simulink model "ElectricVehicleThermalManagementWithHeatPump_2026a_version"  (R2026a)
settings: Solver=VariableStepAuto  StopTime=3600  AbsTol=1e-3
PreLoadFcn:
  | init_nmpc
InitFcn:
  | init_nmpc
model workspace: external: MATLAB File ElectricVehicleThermalManagementWithHeatPumpParameters.m (data not in the file)
values from neighbouring files (symbols this model uses):
  battery_C1_LUT = [1913.6 12447 30609 ... (first row only)    [ElectricVehicleThermalManagementWithHeatPumpParameters.m]
  battery_capacity_LUT = [280.081 276.25 276.392]    [ElectricVehicleThermalManagementWithHeatPumpParameters.m]
  battery_cell_cp = 795    [ElectricVehicleThermalManagementWithHeatPumpParameters.m]
  battery_cell_mass = 2.5    [ElectricVehicleThermalManagementWithHeatPumpParameters.m]
  battery_Em_LUT = [3.4966 3.5057 3.5148 ... (first row only)    [ElectricVehicleThermalManagementWithHeatPumpParameters.m]
  battery_N_cells = 20    [ElectricVehicleThermalManagementWithHeatPumpParameters.m]
  battery_Qe_init = 0    [ElectricVehicleThermalManagementWithHeatPumpParameters.m]
  battery_R0_LUT = [0.0117 0.0085 0.009 ... (first row only)    [ElectricVehicleThermalManagementWithHeatPumpParameters.m]
  battery_R1_LUT = [0.0109 0.0029 0.0013 ... (first row only)    [ElectricVehicleThermalManagementWithHeatPumpParameters.m]
  battery_SOC_LUT = [0; 0.1; 0.25; 0.5; 0.75; 0.9; 1]    [ElectricVehicleThermalManagementWithHeatPumpParameters.m]
  battery_T_init = -5    [ElectricVehicleThermalManagementWithHeatPumpParameters.m]
  battery_temperature_LUT = [5 20 40]    [ElectricVehicleThermalManagementWithHeatPumpParameters.m]
  cabin_duct_area = 0.04    [ElectricVehicleThermalManagementWithHeatPumpParameters.m]
  cabin_T_init = -5    [ElectricVehicleThermalManagementWithHeatPumpParameters.m]
  chiller_area_primary = 0.43982297150257105    (= 0.439822971503)    [ElectricVehicleThermalManagementWithHeatPumpParameters.m]
  chiller_N_baffles = 3    [ElectricVehicleThermalManagementWithHeatPumpParameters.m]
  chiller_N_tubes = 100    [ElectricVehicleThermalManagementWithHeatPumpParameters.m]
  chiller_tube_D = 0.0035    [ElectricVehicleThermalManagementWithHeatPumpParameters.m]
  chiller_tube_L = 0.4    [ElectricVehicleThermalManagementWithHeatPumpParameters.m]
  chiller_wall_conductivity = 240    [ElectricVehicleThermalManagementWithHeatPumpParameters.m]
  chiller_wall_thickness = 0.0001    [ElectricVehicleThermalManagementWithHeatPumpParameters.m]
  cond_evap_air_area_flow = 0.3906    [ElectricVehicleThermalManagementWithHeatPumpParameters.m]
  cond_evap_air_area_primary = 1.4834999999999998    (= 1.4835)    [ElectricVehicleThermalManagementWithHeatPumpParameters.m]
  cond_evap_W = 0.015    [ElectricVehicleThermalManagementWithHeatPumpParameters.m]
  cond_evap_wall_conductivity = 240    [ElectricVehicleThermalManagementWithHeatPumpParameters.m]
  cond_evap_wall_thickness = 0.0001    [ElectricVehicleThermalManagementWithHeatPumpParameters.m]
  coolant_channel_D = 0.0092    [ElectricVehicleThermalManagementWithHeatPumpParameters.m]
  coolant_pipe_D = 0.019    [ElectricVehicleThermalManagementWithHeatPumpParameters.m]
  coolant_T_init = -5    [ElectricVehicleThermalManagementWithHeatPumpParameters.m]
  coolant_tank_area = 0.0121    [ElectricVehicleThermalManagementWithHeatPumpParameters.m]
  coolant_tank_volume = 1.25    [ElectricVehicleThermalManagementWithHeatPumpParameters.m]
  coolant_valve_D_ratio_max = 0.95    [ElectricVehicleThermalManagementWithHeatPumpParameters.m]
  coolant_valve_D_ratio_min = 0.001    [ElectricVehicleThermalManagementWithHeatPumpParameters.m]
  coolant_valve_displacement = 0.0063    [ElectricVehicleThermalManagementWithHeatPumpParameters.m]
  coolant_valve_S_max = 0.0053    [ElectricVehicleThermalManagementWithHeatPumpParameters.m]
  evaporator_air_area_flow = 0.12    [ElectricVehicleThermalManagementWithHeatPumpParameters.m]
  evaporator_air_area_primary = 0.4323    [ElectricVehicleThermalManagementWithHeatPumpParameters.m]
  evaporator_W = 0.015    [ElectricVehicleThermalManagementWithHeatPumpParameters.m]
  evaporator_wall_conductivity = 240    [ElectricVehicleThermalManagementWithHeatPumpParameters.m]
  evaporator_wall_thickness = 0.0001    [ElectricVehicleThermalManagementWithHeatPumpParameters.m]
  expansion_valve_D_ratio_max = 0.9    [ElectricVehicleThermalManagementWithHeatPumpParameters.m]
  hex_area_primary = 0.070371675440411369    (= 0.0703716754404)    [ElectricVehicleThermalManagementWithHeatPumpParameters.m]
  hex_N_tubes = 64    [ElectricVehicleThermalManagementWithHeatPumpParameters.m]
  hex_tube_D = 0.0035    [ElectricVehicleThermalManagementWithHeatPumpParameters.m]
  hex_wall_conductivity = 240    [ElectricVehicleThermalManagementWithHeatPumpParameters.m]
  hex_wall_thickness = 0.0001    [ElectricVehicleThermalManagementWithHeatPumpParameters.m]
  inner_cond_air_area_flow = 0.1953    [ElectricVehicleThermalManagementWithHeatPumpParameters.m]
  inner_cond_air_area_primary = 0.99520000000000008    (= 0.9952)    [ElectricVehicleThermalManagementWithHeatPumpParameters.m]
  inner_cond_W = 0.02    [ElectricVehicleThermalManagementWithHeatPumpParameters.m]
  inner_cond_wall_conductivity = 240    [ElectricVehicleThermalManagementWithHeatPumpParameters.m]
  inner_cond_wall_thickness = 0.0001    [ElectricVehicleThermalManagementWithHeatPumpParameters.m]
  pump_speed_max = 1000    [ElectricVehicleThermalManagementWithHeatPumpParameters.m]
  radiator_air_area_flow = 0.097499999999999989    (= 0.0975)    [ElectricVehicleThermalManagementWithHeatPumpParameters.m]
  radiator_air_area_primary = 0.43687499999999996    (= 0.436875)    [ElectricVehicleThermalManagementWithHeatPumpParameters.m]
  radiator_W = 0.015    [ElectricVehicleThermalManagementWithHeatPumpParameters.m]
  radiator_wall_conductivity = 240    [ElectricVehicleThermalManagementWithHeatPumpParameters.m]
  radiator_wall_thickness = 0.0001    [ElectricVehicleThermalManagementWithHeatPumpParameters.m]
  refrigerant_p_init = 0.25    [ElectricVehicleThermalManagementWithHeatPumpParameters.m]
  refrigerant_pipe_D = 0.01    [ElectricVehicleThermalManagementWithHeatPumpParameters.m]
  refrigerant_valve_D_ratio_max = 0.95    [ElectricVehicleThermalManagementWithHeatPumpParameters.m]
  refrigerant_valve_displacement = 0.005    [ElectricVehicleThermalManagementWithHeatPumpParameters.m]
libraries: fl_lib x227, nesl_utility x162, SimscapeFluids_lib x30, LiBatteryElements_lib x16, slpidlib x3, SignalEditorBlockLib x1
(part 13 of 13)

== matlab function ElectricVehicleThermalManagementWithHeatPump_2026a_version/Controls/MPCControllerBlock/MPCController ==
  data: u_cmd output; x_meas input; Tamb_C input; Tref_K input; clntInvTout_K_meas input; clntBatTin_K_meas input; dcdcQ input; motQ input; invQ input; condEvapAirMf input; batImeas input; info output
function [u_cmd, info] = MPCController_step( ...
    x_meas, ...                         % [nx x 1] measured/estimated states (physical units)
    Tamb_C, ...                         % [1 x 1] ambient in degC
    Tref_K, ...                         % [1 x 1] cabin air reference in K
    clntInvTout_K_meas, ...             % [1 x 1] from plant (K)
    clntBatTin_K_meas, ...              % [1 x 1] from plant (K)
    dcdcQ, motQ, invQ, ...              % [1 x 1] loads (W)
    condEvapAirMf, ...                  % [1 x 1] kg/s
    batImeas)                           % [1 x 1] A
% MPCController_step
% ---------------------------------------------------------
% Simulink usage (continuous plant + discrete MPC):
% - Put MATLAB Function block calling this function in a subsystem with Ts=1
% - ZOH(Ts=1) on u_cmd into continuous plant
% - Rate Transition (to Ts=1) for feedback signals into this block
% - Add Unit Delay(Ts=1) on x_meas path if you get algebraic loop warnings
%
% IMPORTANT:
% This is a "one-step NMPC solve" function. It builds the solver once (persistent),
% then solves once per call and returns the first control move.
%
% NOTE:
% This code keeps your NMPC formulation structure, but to make it deployable in
% a MATLAB Function block, it removes:
% - clc/clear/close
% - any for-loops over ksim (closed-loop simulation loop)
% - any plant rollout inside controller (plant is Simulink)
% ---------------------------------------------------------

%#ok<*NASGU>
%#ok<*AGROW>

% import casadi.*

%% ===================== Persistent objects ============================
persistent built ...
    solver F Uord packParams idx_cmdPS ...
    dt M h N nx nu np ...
    umin umax xmin xmax ...
    Sx SxInv Su SuInv ...
    w_cost w_all p_all g lbg ubg lbw ubw ...
    n_w nX nU nSd idxSdyn idxSy idxSx_lo idxSx_hi ...
    Xsym Usym Sdynsym Sysym Sx_losym Sx_hisym ...
    prev_w_opt prev_lam_x prev_lam_g prev_Pk ...
    inputInit ...
    Stuned resampled ...
    ns_ic idx_ic_slack ...
    USE_FIXED_U USE_SCALING ...
    Tref_default ...
    Gfun

if isempty(built)
    %% =============================== Setup ===============================
    % addpath('C:\Prashant\Prashant\Phd\casadi-3.7.1-windows64-matlab2018b');

    % load('tuning_data_10.mat', 'resampled');
    % tunedVarsFile = 'tunedVariables_minus5_minus10_New.mat';
    % Stuned = load(tunedVarsFile);
    resampled = evalin('base','resampled');
    Stuned    = evalin('base','Stuned');

    [F, Uord, ~, packParams] = create_dynamics_nmpc();
    idx_cmdPS = get_idx_cmdPS(Uord);

    %% ====================== Problem sizes & settings =====================
    dt    = 1.0;     % controller sample time [s]
    M     = 1;       % RK4 sub-steps per sample
    h     = dt/M;
    N     = 30;      % prediction horizon [steps]

    USE_FIXED_U = false;
    USE_SCALING = true;

    %% ============================= Dimensions ============================
    nx = 9;
    nu = numel(Uord.inputSignal);

    %% ====================== Control input bounds =========================
    umin = [    0;   0;    100;   100;   0];
    umax = [ 6000; 0.15; 1000; 1000; 4000];

    %% ====================== State bounds (physical) ======================
    Tmin      = 10 + 273.15;   % K
    Tmax      = 75 + 273.15;   % K
    Pmin      = 0.1e5;         % Pa
    Pmax      = 6e6;           % Pa
    Tmax_cab  = 40 + 273.15;   % K
    Tmin_cab  = 15 + 273.15;  % K
    Tbmin     = 10 + 273.15;   % K
    Tbmax     = 50 + 273.15;   % K

    % [motT; invT; dcdcT; SOC; batT; p_in; p_out; cabIntT; cabAirT]
    xmin = [Tmin; Tmin; Tmin; 0.01; Tbmin; Pmin; Pmin; Tmin_cab; Tmin_cab];
    xmax = [Tmax; Tmax; Tmax; 1.0;  Tbmax; Pmax; Pmax; Tmax_cab; Tmax_cab];

    %% ============================= Scaling ===============================
    sx_data = [max(xmin(1),xmax(1));
               max(xmin(2),xmax(2));
               max(xmin(3),xmax(3));
               max(xmin(4),xmax(4));
               max(xmin(5),xmax(5));
               max(xmin(6),xmax(6));
               max(xmin(7),xmax(7));
               max(xmin(8),xmax(8));
               max(xmin(9),xmax(9))];

    su_data = [ ...
      max(umax(1), max(resampled.compNrpm));
      max(umax(2), max(resampled.cabAirMfIn));
      max(umax(3), max(resampled.motPumpNrpm));
      max(umax(4), max(resampled.motPumpNrpm));
      umax(5)];

    if USE_SCALING
        sx = sx_data(:);
        su = su_data(:);
    else
        sx = ones(nx,1);
        su = ones(nu,1);
    end

    Sx    = diag(sx);
    SxInv = diag(1./sx);
    Su    = diag(su);
    SuInv = diag(1./su);

    physX = @(Xs) Sx*Xs; %#ok<NASGU>

    %% ========================== Weights ==================================
    w = struct();
    w.cab        = 1e1;
    w.cabInt     = 1;
    w.energy     = 1e-3;
    w.du         = 1;
    w.term       = 0.1;
    w.ySlack     = 1e3;
    w.stateSlack = 1e3;

    pwrEstMax   = 11.0e3;
    Q_phys      = zeros(nx);
    Q_phys(9,9) = w.cab;
    Q_s         = Sx.' * Q_phys * Sx;
    R_s         = diag([1e-2, 1e-2, 1e-2, 1e-2, 5e-2]);
    Rd_s        = w.du * eye(nu);

    lambda_du0 = 1;
    lambda_duN = 0.5;
    lambda_du  = linspace(lambda_du0, lambda_duN, N);

    %% ===================== NLP decision variables ========================
    Xsym    = casadi.SX.sym('X',    nx, N+1);    % scaled states
    Sdynsym = casadi.SX.sym('Sdyn', nx, N);      % dynamic slacks (scaled)
    Usym    = casadi.SX.sym('U',    nu, N);      % scaled inputs
    Sysym   = casadi.SX.sym('S_y',  3,  N);      % inequality slacks (free in your script)

    idx_ic_slack = [1; 2; 3; 5; 8; 9];
    ns_ic        = numel(idx_ic_slack);
    Sx_losym     = casadi.SX.sym('Sx_lo', ns_ic, N+1);
    Sx_hisym     = casadi.SX.sym('Sx_hi', ns_ic, N+1);

    % Parameters (physical)
    p_x0          = casadi.SX.sym('p_x0',   nx, 1);
    p_Tref        = casadi.SX.sym('p_Tref', 1,  N+1);

    % ---- pack stage params size using one sample ----
    % We will determine np after first thermalLogic call at runtime too,
    % but here we build a dummy np by doing a "local" numeric call once.
    % (We do a safe default and then overwrite np later if needed.)
    % We'll set np after creating p_sample below.

    % We'll define Pstage later after np is known.
    % For building the NLP we need np now => do a dummy call:
    Tamb0 = -10;
    x0_dummy = [ ...
        20+273.15; 20+273.15; 20+273.15; 0.8; 20+273.15; ...
        2e5; 3e6; 20+273.15; 20+273.15];
    inputInit0.envT          = Tamb0 + 273.15;
    inputInit0.clntInvTout_K = Tamb0 + 273.15;
    inputInit0.clntBatTin_K  = Tamb0 + 273.15;
    inputInit0.compN         = 0;
    inputInit0.pumpN         = 100;
    inputInit0.prevMode      = 0;
    inputInit0.heaterPwr     = 0;

    heat0.dcdcQ         = 0;
    heat0.motQ          = 0;
    heat0.invQ          = 0;
    heat0.condEvapAirMf = 0.05;
    heat0.batImeas      = 0;
    heat0.superHeat     = 2;

    tuneS0 = prepParaVec(x0_dummy, Tamb0, Stuned.tunedVariables);
    [ctrl0, est0] = thermalLogicAndEstimation(x0_dummy, inputInit0, heat0);
    p_sample      = packParams(est0, ctrl0, tuneS0);
    np            = numel(p_sample);

    Pstage        = casadi.SX.sym('Pstage', np, N);
    p_u_last_phys = casadi.SX.sym('p_u_last_phys', nu, 1);

    % Terminal terms: keep them but lightweight default P=I, xT=x0, uT=u_last
    p_xT = casadi.SX.sym('p_xT', nx, 1);
    p_uT = casadi.SX.sym('p_uT', nu, 1);
    p_P  = casadi.SX.sym('p_P',  nx*nx, 1);   % vec(P)

    p_all = vertcat(p_x0, p_Tref(:), Pstage(:), p_xT, p_uT, p_P, p_u_last_phys);

    %% ============================ Objective/Constraints ==================
    w_cost = 0;
    g      = {};
    lbg    = [];
    ubg    = [];

    % Reference in scaled space
    Xref_s      = casadi.SX.zeros(nx, N+1);
    Xref_s(9,:) = p_Tref / Sx(9,9);

    % IC equality: X(:,1) = p_x0
    r0_phys   = Sx*Xsym(:,1) - p_x0;
    r0_scaled = SxInv * r0_phys;
    for i = 1:nx
        g{end+1} = r0_scaled(i);
        lbg      = [lbg; 0];
        ubg      = [ubg; 0];
    end

    % Slack penalties
    w_cost = w_cost + w.ySlack * sum1(Sysym(:).^2);
    w_cost = w_cost + w.stateSlack * ( sum1(Sx_losym(:).^2) + sum1(Sx_hisym(:).^2) );

    % Some constants used in your constraints
    clntLow  = -51+273.15;
    clntHigh = 121+273.15;

    rho_dyn2   = 5e3;
    rho_dyn1   = 1e1;

    % Dynamics + stage cost
    for k = 1:N
        xk_phys = Sx*Xsym(:,k);
        pk      = Pstage(:,k);
        Uk_phys = Su*Usym(:,k);

        % RK4
        xtmp = xk_phys;
        for j = 1:M
            [xdot1, ~, ~] = F(xtmp,               Uk_phys, pk);
            [xdot2, ~, ~] = F(xtmp + 0.5*h*xdot1, Uk_phys, pk);
            [xdot3, ~, ~] = F(xtmp + 0.5*h*xdot2, Uk_phys, pk);
            [xdot4, ~, ~] = F(xtmp +     h*xdot3, Uk_phys, pk);
            xtmp = xtmp + h/6*(xdot1 + 2*xdot2 + 2*xdot3 + xdot4);
        end

        [~, ~, pwr] = F(xtmp, Uk_phys, pk);

        % Dynamics constraints
        rk_scaled = SxInv * (Sx*Xsym(:,k+1) - xtmp);
        g{end+1}  = rk_scaled - Sdynsym(:,k);
        lbg       = [lbg; zeros(nx,1)];
        ubg       = [ubg; zeros(nx,1)];

        % Dynamic slack penalties + power
        eps_s   = 1e-5;
        Sdyn_k  = Sdynsym(:,k);
        w_cost  = w_cost + rho_dyn2*sumsqr(Sdyn_k) + rho_dyn1*sum1(sqrt(Sdyn_k.^2 + eps_s)) + pwr./pwrEstMax;

        % State tracking
        eXk = Xsym(:,k) - Xref_s(:,k);
        w_cost = w_cost + eXk.'*Q_s*eXk;

        % Parallel/serial mode constraint: mPS*(U3-U4)=0
        mPS = Pstage(idx_cmdPS, k);
        g{end+1} = mPS * (Usym(3,k) - Usym(4,k));
        lbg      = [lbg; 0];
        ubg      = [ubg; 0];

        % Input penalties + slew penalties
        Uk_s = Usym(:,k);
        w_cost = w_cost + Uk_s.' * R_s * Uk_s;

        if k == 1
            dUk_s = Usym(:,1) - (SuInv * p_u_last_phys);
        else
            dUk_s = Usym(:,k) - Usym(:,k-1);
        end
        w_cost = w_cost + lambda_du(k) * (dUk_s.' * Rd_s * dUk_s);

        % Algebraic outputs for your constraints
        [~, yavg_k, ~] = F(xtmp, Uk_phys, pk);
        innerCondRefToutK = yavg_k(10);
        innerCondAirTinK  = yavg_k(27);
        htxClntToutK      = yavg_k(6);
        refTempCompInK    = yavg_k(14);
        invClntToutK      = yavg_k(1);
        motClntToutK      = yavg_k(2);
        dcdcClntToutK     = yavg_k(5);
        heaterClntToutK   = yavg_k(7);
        heaterClntTInK    = yavg_k(30);

        Sy1k = Sysym(1,k);
        Sy2k = Sysym(2,k);
        Sy3k = Sysym(3,k);

        % innerCondRefToutK >= innerCondAirTinK (with slack)
        g{end+1} = innerCondRefToutK - innerCondAirTinK + Sy1k;
        lbg      = [lbg; 0];
        ubg      = [ubg; inf];

        % heater deltaT constraint
        dT_heater_max = 18;
        g{end+1} = heaterClntToutK - heaterClntTInK;
        lbg      = [lbg; -inf];
        ubg      = [ubg; dT_heater_max];

        % superheat-ish constraint (your #3)
        g{end+1} = (Pstage(38,k) + 2) - refTempCompInK + Sy3k;
        lbg      = [lbg; -2];
        ubg      = [ubg; 10];

        % coolant bounds
        g{end+1} = htxClntToutK;    lbg=[lbg;clntLow];  ubg=[ubg;clntHigh];
        g{end+1} = heaterClntToutK; lbg=[lbg;clntLow];  ubg=[ubg;clntHigh];
        g{end+1} = invClntToutK;    lbg=[lbg;clntLow];  ubg=[ubg;clntHigh];
        g{end+1} = motClntToutK;    lbg=[lbg;clntLow];  ubg=[ubg;clntHigh];
        g{end+1} = dcdcClntToutK;   lbg=[lbg;clntLow];  ubg=[ubg;clntHigh];
    end

    % Soft bounds over horizon for selected states
    for k = 1:(N+1)
        xk_phys = Sx*Xsym(:,k);
        for j = 1:ns_ic
            i   = idx_ic_slack(j);
            slo = Sx_losym(j,k);
            shi = Sx_hisym(j,k);

            g{end+1} = xmin(i) - xk_phys(i) - slo;   lbg=[lbg;-inf]; ubg=[ubg;0];
            g{end+1} = xk_phys(i) - xmax(i) - shi;   lbg=[lbg;-inf]; ubg=[ubg;0];
        end
    end

    % Terminal cost: (X(N+1)-xT)'*P*(X(N+1)-xT) + small tie-to-uT
    Pmat  = reshape(p_P, nx, nx);
    eXN   = Xsym(:,N+1) - (SxInv*p_xT);
    w_cost = w_cost + eXN.'*Pmat*eXN;
    uT_s   = SuInv * p_uT;
    w_cost = w_cost + 1e-3 * (Usym(:,N) - uT_s).'*R_s*(Usym(:,N) - uT_s);

    % Pack decision variables
    w_all = [Xsym(:); Usym(:); Sdynsym(:); Sysym(:); Sx_losym(:); Sx_hisym(:)];

    % Bounds
    lbw = -inf(size(w_all));
    ubw = +inf(size(w_all));

    % Hard state box bounds (scaled) for all nodes (then relaxed on slacked indices)
    xmin_s = SxInv * xmin;
    xmax_s = SxInv * xmax;
    for k = 1:(N+1)
        i0 = (k-1)*nx;
        lbw(i0 + (1:nx)) = xmin_s;
        ubw(i0 + (1:nx)) = xmax_s;
    end

    % Relax slacked temperature states to very wide hard bounds
    Tlo_hard = (-60 + 273.15);
    Thi_hard = (140 + 273.15);
    for k = 1:(N+1)
        i0 = (k-1)*nx;
        for kk = 1:ns_ic
            ii = idx_ic_slack(kk);
            lbw(i0 + ii) = Tlo_hard / sx(ii);
            ubw(i0 + ii) = Thi_hard / sx(ii);
        end
    end

    % Input bounds (scaled)
    umin_s = SuInv * umin;
    umax_s = SuInv * umax;
    offU = numel(Xsym(:));
    for k = 1:N
        u0 = offU + (k-1)*nu;
        lbw(u0 + (1:nu)) = umin_s;
        ubw(u0 + (1:nu)) = umax_s;
    end

    % Index layout
    nX   = numel(Xsym(:));
    nU   = numel(Usym(:));
    nSd  = nx*N;
    idxSdyn  = nX + nU + (1:nSd);

    nSy   = 3*N;
    idxSy = nX + nU + nSd + (1:nSy);

    nSx      = ns_ic*(N+1);
    idxSx_lo = nX + nU + nSd + nSy + (1:nSx);
    idxSx_hi = nX + nU + nSd + nSy + nSx + (1:nSx);

    % Bounds for Sx slacks
    lbw(idxSx_lo) = 0; ubw(idxSx_lo) = inf;
    lbw(idxSx_hi) = 0; ubw(idxSx_hi) = inf;

    % Bounds for S_y (your script allows negative, but you clamp later)
    lbw(idxSy) = -1000; ubw(idxSy) = 1000;

    % Bounds for Sdyn: allow free (you were not strictly bounding in scaled case)
    lbw(idxSdyn) = -inf;
    ubw(idxSdyn) =  inf;

    % Constraint function for debug (optional)
    Gfun = casadi.Function('Gfun', {w_all, p_all}, {vertcat(g{:})});

    % NLP
    prob = struct('f', w_cost, 'x', w_all, 'g', vertcat(g{:}), 'p', p_all);

    % Solver options (your robust-ish setup)
    opts = struct;
    opts.error_on_fail      = false;
    opts.print_time         = false;
    opts.ipopt.max_iter     = 2000;
    opts.ipopt.tol          = 1e-3;
    opts.ipopt.constr_viol_tol  = 1e-5;
    opts.ipopt.dual_inf_tol     = 1e-3;
    opts.ipopt.compl_inf_tol    = 1e-3;
    opts.ipopt.hessian_approximation = 'exact';
    opts.ipopt.linear_solver     = 'mumps';
    opts.ipopt.mu_strategy       = 'adaptive';
    opts.ipopt.print_level       = 0;   % set 5 if you want logs (but Simulink will spam)
    opts.calc_lam_p              = true;

    solver = casadi.nlpsol('solver', 'ipopt', prob, opts);

    % Persistent memory init
    prev_w_opt = [];
    prev_lam_x = [];
    prev_lam_g = [];

    inputInit.envT          = (Tamb_C + 273.15);
    inputInit.clntInvTout_K = (Tamb_C + 273.15);
    inputInit.clntBatTin_K  = (Tamb_C + 273.15);
    inputInit.compN         = 0;
    inputInit.pumpN         = 100;
    inputInit.prevMode      = 0;
    inputInit.heaterPwr     = 0;

    prev_Pk = repmat(p_sample, 1, N);

    Tref_default = 294.15;

    built = true;
end

%% ===================== Per-step MPC solve ============================
% Update supervisor “memory” from plant (Option P1)
inputInit.clntInvTout_K = clntInvTout_K_meas;
inputInit.clntBatTin_K  = clntBatTin_K_meas;
inputInit.envT          = Tamb_C + 273.15;

% Build horizon measurement struct (simple: hold current across horizon)
heatMeasured_k.dcdcQ         = repmat(dcdcQ, N, 1);
heatMeasured_k.motQ          = repmat(motQ,  N, 1);
heatMeasured_k.invQ          = repmat(invQ,  N, 1);
heatMeasured_k.condEvapAirMf = repmat(max(condEvapAirMf,1e-5), N, 1);
heatMeasured_k.batImeas      = repmat(max(batImeas,1e-3), N, 1);
heatMeasured_k.superHeat     = 2;

% Tune + supervisor/estimation
tuneS = prepParaVec(x_meas, Tamb_C, Stuned.tunedVariables);
[ctrl, est] = thermalLogicAndEstimation(x_meas, inputInit, heatMeasured_k);

% Pack stage params Pk
Pk = zeros(np, N);
for i = 1:N
    est_i = est;

    % overwrite stage-varying measured quantities if fields exist
    if isfield(est_i,'condEvapAirMf'), est_i.condEvapAirMf = heatMeasured_k.condEvapAirMf(i); end
    if isfield(est_i,'batImeas'),      est_i.batImeas      = heatMeasured_k.batImeas(i);      end
    if isfield(est_i,'motQmeas'),      est_i.motQmeas      = heatMeasured_k.motQ(i);          end
    if isfield(est_i,'invQmeas'),      est_i.invQmeas      = heatMeasured_k.invQ(i);          end
    if isfield(est_i,'dcdcQmeas'),     est_i.dcdcQmeas     = heatMeasured_k.dcdcQ(i);         end
    if isfield(est_i,'superheatK'),    est_i.superheatK    = heatMeasured_k.superHeat;        end

    pk_col = packParams(est_i, ctrl, tuneS);
    if ~all(isfinite(pk_col))
        pk_col = prev_Pk(:,i);
    end
    Pk(:,i) = pk_col;
end
prev_Pk = Pk;

% Reference path
if isempty(Tref_K) || ~isfinite(Tref_K)
    Tref_K = Tref_default;
end
Tref_path = Tref_K * ones(N+1,1);

% Terminal placeholders (lightweight but keeps your p_all format consistent)
xT    = x_meas;
uT    = [inputInit.compN; 0.05; inputInit.pumpN; inputInit.pumpN; inputInit.heaterPwr];
Pterm = eye(nx);

% Previous applied u (persistent)
persistent u_last
if isempty(u_last)
    u_last = uT;
end

% pvec must match p_all = [x0; Tref; Pstage(:); xT; uT; vec(P); u_last]
pvec = [x_meas; Tref_path; Pk(:); xT; uT; Pterm(:); u_last];

% Build warm start w0
w0 = zeros(n_w,1);

% states init guess: keep constant (scaled)
Xs0 = repmat(SxInv*x_meas, 1, N+1);
w0(1:nX) = Xs0(:);

% inputs init guess: keep last u (scaled)
Us0 = repmat(SuInv*u_last, 1, N);
w0(nX + (1:nU)) = Us0(:);

% slacks init guess: zeros but make soft-bound slacks feasible
w0(idxSdyn)  = 0;
w0(idxSy)    = 0;

% compute soft slacks for current X guess
Xphys0 = Sx * reshape(w0(1:nX), nx, N+1);
Sx_lo0 = zeros(ns_ic, N+1);
Sx_hi0 = zeros(ns_ic, N+1);
for kk = 1:(N+1)
    for j = 1:ns_ic
        ii = idx_ic_slack(j);
        Sx_lo0(j,kk) = max(0, xmin(ii) - Xphys0(ii,kk));
        Sx_hi0(j,kk) = max(0, Xphys0(ii,kk) - xmax(ii));
    end
end
w0(idxSx_lo) = Sx_lo0(:);
w0(idxSx_hi) = Sx_hi0(:);

% Shift warm start from previous solve if available
if ~isempty(prev_w_opt)
    w0 = shift_warm_start_full(prev_w_opt, w0, nx, nu, N, nX, nU, idxSdyn, idxSy, idxSx_lo, idxSx_hi);
end

% Solve
args = {'x0', w0, ...
        'lbx', lbw, 'ubx', ubw, ...
        'lbg', lbg, 'ubg', ubg, ...
        'p',   pvec};

if ~isempty(prev_lam_x), args(end+1:end+2) = {'lam_x0', prev_lam_x}; end
if ~isempty(prev_lam_g), args(end+1:end+2) = {'lam_g0', prev_lam_g}; end

sol = solver(args{:});
st  = solver.stats();

w_opt = full(sol.x);

% Extract first move
U_opt_s = reshape(w_opt(nX + (1:nU)), nu, N);
u_cmd   = Su * U_opt_s(:,1);

% Update warm-start memory
prev_w_opt = w_opt;
if isfield(sol,'lam_x'), prev_lam_x = full(sol.lam_x); else, prev_lam_x = []; end
if isfield(sol,'lam_g'), prev_lam_g = full(sol.lam_g); else, prev_lam_g = []; end

% Update controller memory for next call
inputInit.compN     = u_cmd(1);
inputInit.pumpN     = u_cmd(3);
inputInit.heaterPwr = u_cmd(5);
if isfield(ctrl,'thermalMode')
    inputInit.prevMode = ctrl.thermalMode;
end
u_last = u_cmd;

% Info
info.success = logical(st.success);
if isfield(st,'iter_count'), info.iter = double(st.iter_count); else, info.iter = NaN; end
if isfield(st,'return_status'), info.status = string(st.return_status); else, info.status = ""; end
info.obj = full(sol.f);

end

%% ============================ Helpers ===============================

function w0_next = shift_warm_start_full(prev_w_opt, w0, nx, nu, N, nX, nU, idxSdyn, idxSy, idxSx_lo, idxSx_hi)
    % shift X
    Xs  = reshape(prev_w_opt(1:nX), nx, N+1);
    Xs_shift = [Xs(:,2:end), Xs(:,end)];
    w0_next = w0;
    w0_next(1:nX) = Xs_shift(:);

    % shift U
    Us = reshape(prev_w_opt(nX + (1:nU)), nu, N);
    Us_shift = [Us(:,2:end), Us(:,end)];
    w0_next(nX + (1:nU)) = Us_shift(:);

    % shift Sdyn
    Sd = reshape(prev_w_opt(idxSdyn), nx, N);
    Sd_shift = [Sd(:,2:end), Sd(:,end)];
    w0_next(idxSdyn) = Sd_shift(:);

    % keep Sy, Sx_lo, Sx_hi
    w0_next(idxSy)    = prev_w_opt(idxSy);
    w0_next(idxSx_lo) = prev_w_opt(idxSx_lo);
    w0_next(idxSx_hi) = prev_w_opt(idxSx_hi);
end

function idx = get_idx_cmdPS(Uord)
    names = [Uord.estimatedParams(:); Uord.controlOut(:); Uord.tunePara(:)];
    idx   = find(strcmp(names, 'cmdParallelSerial'), 1);
    if isempty(idx)
        error('cmdParallelSerial not found in packParams order.');
    end
end

== matlab function ElectricVehicleThermalManagementWithHeatPump_2026a_version/Scenario/Power Demand/MATLAB Function ==
  data: OCV output; negSide output; speed_kph input; acceleration_current input size=1; road_grade input; lossTq output; lossInv output; lossDCDC output; battery_current output; Total_power output; U_lo input; U_hi input; power_motor_electrical_input output; blowerVF input; motPumpPwr input; SOC input; batTemp input; prevBatTemp input
function [OCV, negSide, lossTq, lossInv, lossDCDC, battery_current, Total_power, power_motor_electrical_input] = pwrEstimation(speed_kph, acceleration_current, road_grade, U_lo, U_hi, blowerVF, motPumpPwr, SOC, batTemp, prevBatTemp)
% =========================================================================
% Electric Motor and Battery Estimation Model (Simulink MATLAB Function)
% =========================================================================
% This function estimates:
%   - Electric motor torque and speed
%   - Motor, inverter, and DC-DC converter power losses
%   - Battery power demand and current using an Equivalent Circuit Model (ECM)
%
% -------------------------------------------------------------------------
% Author        : Prashant Lokur
% Affiliation   : Chalmers University of Technology
% Contact       : lokur@chalmers.se
% Created       : 2024
%
% Copyright (c) 2024 Prashant Lokur
% All rights reserved.
%
% This code is intended for academic and research use only.
% Redistribution and use in source and binary forms, with or without
% modification, are permitted provided that the above attribution is retained.
%
% For inquiries regarding licensing for commercial or industrial applications,
% please contact the author.

% This function estimates:
%   - Electric motor torque and speed
%   - Losses in motor, inverter, and DC-DC converter
%   - Battery current using an Equivalent Circuit Model (ECM)
% 
% Inputs:
%   speed_kph         - Vehicle speed (km/h)
%   acceleration_current - Vehicle acceleration (m/s^2)
%   road_grade        - Road slope in percentage (%)
%   U_lo, U_hi        - Low and high voltages of the DCDC converter (V)
%   blowerVF          - Blower voltage fraction (0 to 1)
%   motPumpPwr        - Motor pump power consumption (W)
%   SOC               - Battery State of Charge (0 to 1)
%   batTemp           - Current battery temperature (°C)
%   prevBatTemp       - Previous battery temperature used if current is invalid
%
% Outputs:
%   OCV                      - Battery open circuit voltage (V)
%   negSide                  - Intermediate calculation: -4*P_demand*R0 (for diagnostics)
%   power_motor_mechanical_output - Power at the motor shaft (W)
%   lossTq                  - Motor loss (W)
%   lossInv                 - Inverter loss (W)
%   lossDCDC                - DC-DC converter loss (W)
%   battery_current         - Estimated battery current (A)
%   Total_power             - Total battery power demand (W)
%   power_motor_electrical_input - Motor electrical input power (W)

% =========================================================================
% SECTION 1: Data Preprocessing and Constants
% =========================================================================

% Replace invalid battery temperature with previous value
if batTemp < -50 || batTemp > 150 || isnan(batTemp)
    batTemp = prevBatTemp;
end

% Constants
g = 9.81;                 % Gravity (m/s^2)
rho_air = 1.225;          % Air density (kg/m^3)
Crr = 0.015;              % Rolling resistance coefficient
Cd = 0.3;                 % Drag coefficient
wheel_radius = 0.3;       % Wheel radius (m)
gear_ratio = 8;           % Gear ratio (motor speed / wheel speed)
gear_efficiency = 0.98;   % Gear efficiency
vehicle_mass = 1200;      % Vehicle mass (kg)
frontal_area = 2;         % Frontal area (m^2)

% Convert speed to m/s
speed_mps = speed_kph * 1000 / 3600;
theta_road = atan(road_grade / 100);

% =========================================================================
% SECTION 2: Force and Power Calculations
% =========================================================================

F_rr = Crr * vehicle_mass * g * cos(theta_road);                  % Rolling resistance
F_drag = 0.5 * rho_air * Cd * frontal_area * speed_mps^2;         % Aerodynamic drag
F_gravity = vehicle_mass * g * sin(theta_road);                   % Grade force
F_inertia = vehicle_mass * acceleration_current;                  % Inertial force
F_total = F_rr + F_drag + F_gravity + F_inertia;                  % Total traction force

power_wheel = F_total * speed_mps;                                % Power at the wheels

omega_motor_rad_s = (speed_mps / wheel_radius) * gear_ratio;      % Motor speed (rad/s)
omega_motor_rpm_out = omega_motor_rad_s * (60 / (2 * pi));        % Motor speed (RPM)

torque_wheel = F_total * wheel_radius;                            % Wheel torque
torque_motor_out = torque_wheel / (gear_ratio * gear_efficiency); % Motor torque

% =========================================================================
% SECTION 3: Motor Loss Estimation
% =========================================================================

persistent MotorLossData DataLoadedMotor
if isempty(DataLoadedMotor)
    MotorLossData = load('motLoss.mat');
    DataLoadedMotor = true;
    [MotorLossData.omega, idx_omega] = sort(MotorLossData.omega);
    [MotorLossData.Tq, idx_tq] = sort(MotorLossData.Tq);
    MotorLossData.loss = MotorLossData.loss(idx_tq, :);
    MotorLossData.loss = MotorLossData.loss(:, idx_omega);
end

omega_interp = min(max(omega_motor_rpm_out, min(MotorLossData.omega)), max(MotorLossData.omega));
torque_interp = min(max(torque_motor_out, min(MotorLossData.Tq)), max(MotorLossData.Tq));

lossTq = interp2(MotorLossData.omega, MotorLossData.Tq, MotorLossData.loss, omega_interp, torque_interp, 'linear', 0);

% =========================================================================
% SECTION 4: Inverter Loss Estimation
% =========================================================================

persistent InverterLossData DataLoadedInverter
if isempty(DataLoadedInverter)
    InverterLossData = load('invLoss.mat');
    DataLoadedInverter = true;
    [InverterLossData.invOmega, idx_omega] = sort(InverterLossData.invOmega);
    [InverterLossData.invTq, idx_tq] = sort(InverterLossData.invTq);
    InverterLossData.invLoss = InverterLossData.invLoss(idx_tq, :);
    InverterLossData.invLoss = InverterLossData.invLoss(:, idx_omega);
end

omega_interp_inv = min(max(omega_motor_rpm_out, min(InverterLossData.invOmega)), max(InverterLossData.invOmega));
torque_interp_inv = min(max(torque_motor_out, min(InverterLossData.invTq)), max(InverterLossData.invTq));

lossInv = interp2(InverterLossData.invOmega, InverterLossData.invTq, InverterLossData.invLoss, omega_interp_inv, torque_interp_inv, 'linear', 0);

% =========================================================================
% SECTION 5: Battery Open Circuit Voltage and R0 (LUT)
% =========================================================================
  % Battery Look-Up Tables (LUTs)
    battery_Em_LUT = ...        % Open circuit Voltage (V) vs SOC and Temperature
      [3.4966 3.5057 3.5148;
       3.5519 3.566 3.5653;
       3.6183 3.6337 3.6402;
       3.7066 3.7127 3.7213;
       3.9131 3.9259 3.9376;
       4.0748 4.0777 4.0821;
       4.1923 4.1928 4.193];
    battery_capacity_LUT = [280.081 276.25 276.392]; % Battery capacity (Ah) vs Temperature
    battery_R0_LUT = ...        % Battery internal resistance (Ohm) vs SOC and Temperature
      [0.0117 0.0085 0.009;
       0.011 0.0085 0.009;
       0.0114 0.0087 0.0092;
       0.0107 0.0082 0.0088;
       0.0107 0.0083 0.0091;
       0.0113 0.0085 0.0089;
       0.0116 0.0085 0.0089];
    battery_SOC_LUT = [0; 0.1; 0.25; 0.5; 0.75; 0.9; 1]; % SOC values for LUTs
    battery_temperature_LUT = [278.15, 293.15, 313.15]; % Temperature values for LUTs (K)

OCV = interp2(battery_temperature_LUT, battery_SOC_LUT, battery_Em_LUT, batTemp+273.15, SOC, 'spline') * 4 * 30;
batR0 = interp2(battery_temperature_LUT, battery_SOC_LUT, battery_R0_LUT, batTemp+273.15, SOC, 'spline');

% =========================================================================
% SECTION 6: DC-DC Converter Loss Estimation
% =========================================================================

blowerPower_W = 182.3651*blowerVF^2 - 4.9622*blowerVF + 0.0793;
Pwr_dcdc = blowerPower_W + 2 * motPumpPwr;

Vce = 0.7552; rce = 0.8356e-3; Vd0 = 0.8812; rd0 = 1.143e-3;
Esw = 0.04149; Erec = 0.006182; fsw = 20000;
Unom = 400; Inom = 450;

Idcdc_lo = Pwr_dcdc / U_lo;
d = U_hi / U_lo;

Pcond = (Vce*Idcdc_lo + rce*Idcdc_lo^2)*d + (Vd0*Idcdc_lo + rd0*Idcdc_lo^2)*(1-d);
Psw = Esw*U_hi*Idcdc_lo/(pi*Inom*Unom)*fsw + Erec*U_hi*Idcdc_lo/(pi*Inom*Unom)*fsw;

lossDCDC = Pcond + Psw;

% =========================================================================
% SECTION 7: Battery Power Demand and Current Estimation
% =========================================================================

power_motor_mechanical_output = power_wheel / gear_efficiency;
power_motor_electrical_input = (torque_interp * omega_interp) * 2*pi/60 + lossTq;
battery_power_demand = power_motor_electrical_input + lossInv + lossDCDC + Pwr_dcdc;
Total_power = battery_power_demand;

% Quadratic Equation: R0*I^2 - Voc*I + P = 0
a = batR0;
b = -OCV;
c = battery_power_demand;
discriminant = b^2 - 4*a*c;

negSide = -4 * battery_power_demand * batR0;

% if discriminant >= 0
%     i1 = (-b + sqrt(discriminant)) / (2*a);
%     i2 = (-b - sqrt(discriminant)) / (2*a);
%     battery_current = min([i1 i2 i1>=0 i2>=0]*[1;1;0;0]); % Smallest non-negative
% else
%     battery_current = 0;
%     disp('Warning: No real solution for battery current. Power demand might be too high or ECM parameters invalid.');
% end

% Alternative approach used for ECM-based current:
batteryCcurrent = 1/(2*a)*(OCV - sqrt(max(0, OCV^2 - 4*a*c)));
battery_current = batteryCcurrent;

end

== matlab function ElectricVehicleThermalManagementWithHeatPump_2026a_version/Controls/Preview/SpeedPreview ==
  data: t input; v_vec output size=N; t_grid input; v_grid input; a_vec output size=N; a_grid input; tenv input; Tenv_vec output size=N
function [v_vec, a_vec, Tenv_vec] = SpeedPreview(t, t_grid, v_grid, a_grid, tenv)
%#codegen
% Output size is always N_MAX x 1 — completely fixed, no parameters needed.
% Downstream blocks always receive N_MAX elements.
% N_MAX must match the value set in init_nmpc.m

%% ── ONLY line to change when N changes ───────────────────────────────────
N_MAX = 30;   % ← hardcoded compile-time constant, must match init_nmpc N

%% ── Fixed-size outputs (N_MAX is a literal — codegen has no ambiguity) ───
v_vec    = zeros(N_MAX, 1);
a_vec    = zeros(N_MAX, 1);
Tenv_vec = zeros(N_MAX, 1);

%% ── Sample time (hardcoded for same reason) ──────────────────────────────
Ts_val = 1.0;   % ← must match init_nmpc Ts

%% ── Grid info ────────────────────────────────────────────────────────────
t0 = t_grid(1);
t1 = t_grid(end);
m  = numel(t_grid);

%% ── Per-step interpolation ───────────────────────────────────────────────
for i = 1:N_MAX

    % Preview time for step i, clamped to grid range
    tau_i = t + (double(i) - 1.0) * Ts_val;
    if tau_i < t0
        tau_i = t0;
    elseif tau_i > t1
        tau_i = t1;
    end

    % Binary search for bracketing index
    lo = 1;
    hi = m - 1;
    while lo < hi
        mid = floor((lo + hi) / 2);
        if t_grid(mid + 1) <= tau_i
            lo = mid + 1;
        else
            hi = mid;
        end
    end
    idx = lo;

    % Interpolation weight
    dt_seg = t_grid(idx+1) - t_grid(idx);
    if dt_seg > 0.0
        w = (tau_i - t_grid(idx)) / dt_seg;
    else
        w = 0.0;
    end
    w = max(0.0, min(1.0, w));   % clamp weight to [0,1]

    % Write directly into pre-allocated fixed arrays
    v_vec(i)    = (1.0 - w) * v_grid(idx) + w * v_grid(idx + 1);
    a_vec(i)    = (1.0 - w) * a_grid(idx) + w * a_grid(idx + 1);
    Tenv_vec(i) = tenv;
end

end

== matlab function ElectricVehicleThermalManagementWithHeatPump_2026a_version/Condenser Evaporator/MATLAB Function ==
  data: u input; y output
function y = fcn(u)
y = 0.4821*0.04*1.34*u/3.6;

== matlab function ElectricVehicleThermalManagementWithHeatPump_2026a_version/Controls/Preview/condEvapAirFlow2 ==
  data: speed input; mfCondEvap output size=[N 1]
function mfCondEvap = fcn(speed)
mfCondEvap = 0.4821*0.04*1.34*speed/3.6;

end
